simulink model "walec_ostroslup_simulink"  (R2025b)
settings: Solver=FixedStepAuto  StartTime=0.0  StopTime=100  FixedStep=0.0001  RelTol=1e-3
values from neighbouring files (symbols this model uses):
  A2 = 1.47044    [PA_Lab4_walec_ostroslup.m]
  B2 = 4.08042    [PA_Lab4_walec_ostroslup.m]
  C1 = 1.8257    [PA_Lab4_walec_ostroslup.m]
  C2 = 0.745356    [PA_Lab4_walec_ostroslup.m]
  dw = 0.1    [PA_Lab4_walec_ostroslup.m]
  h10 = (qwe0/C1)^2    [PA_Lab4_walec_ostroslup.m]
  H2 = 10    [PA_Lab4_walec_ostroslup.m]
  h20 = 0.5*H2    (= 5)    [PA_Lab4_walec_ostroslup.m]
  kr = 1.2*T_nl/(k_nl*To_nl)    [PA_Lab4_walec_ostroslup.m]
  qwe0 = C2*sqrt(h20)    [PA_Lab4_walec_ostroslup.m]
  R1 = 1.9544    [PA_Lab4_walec_ostroslup.m]
settings Model: Creator=Matadoo  LastModifiedBy=wystr

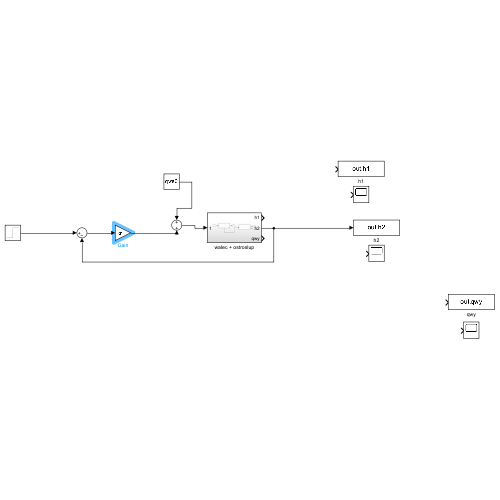
[thumbnail: Simulink's stored preview of the top-level diagram]
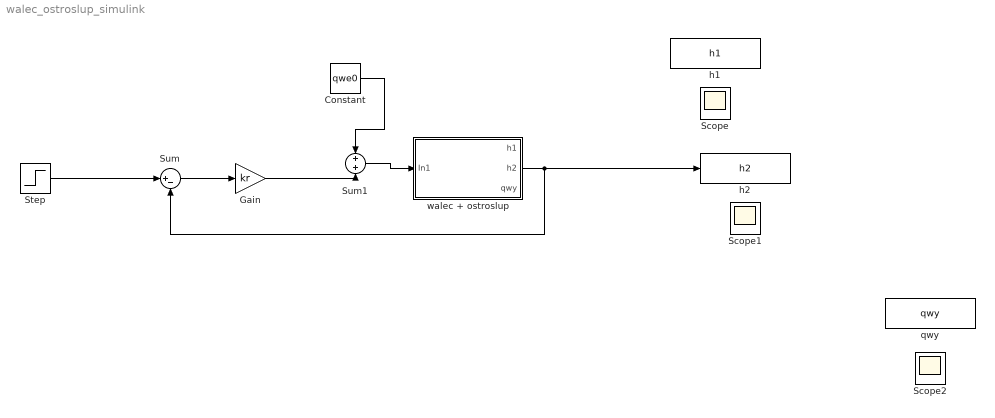
== system walec_ostroslup_simulink ==
  Constant : Constant  Value=qwe0
  Gain : Gain  Gain=kr
  Scope : Scope
      settings: ActiveDisplayYMinimum=-1  ActiveDisplayYMaximum=1
  Scope1 : Scope
      settings: ActiveDisplayYMinimum=0.54521  ActiveDisplayYMaximum=9.07763
  Scope2 : Scope
      settings: ActiveDisplayYMinimum=-1  ActiveDisplayYMaximum=1  DataLoggingVariableName=ScopeData2
  Step : Step  Time=0  Before=h20  After=h20 + dw  SampleTime=0
  Sum : Sum  Inputs=|+-
  Sum1 : Sum  Inputs=+|+
  h1 : ToWorkspace  VariableName=h1  SaveFormat=Timeseries  SampleTime=-1
      settings: Save2DSignal=2-D array (concatenate along first dimension)
  h2 : ToWorkspace  VariableName=h2  SaveFormat=Timeseries  SampleTime=-1
      settings: Save2DSignal=2-D array (concatenate along first dimension)
  qwy : ToWorkspace  VariableName=qwy  SaveFormat=Timeseries  SampleTime=-1
      settings: Save2DSignal=2-D array (concatenate along first dimension)
  walec + ostroslup : Subsystem
  wires:
  walec + ostroslup/2(h2) -> h2/1, Sum/2
  Step/1 -> Sum/1
  Sum/1 -> Gain/1
  Constant/1 -> Sum1/1
  Gain/1 -> Sum1/2
  Sum1/1 -> walec + ostroslup/1(In1)

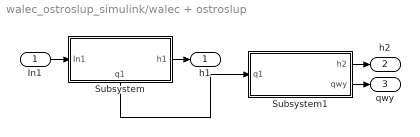
== system walec_ostroslup_simulink/walec + ostroslup ==
  In1 : Inport
  Subsystem : Subsystem
      settings: PortSchema="{\"entries\":[{\"content\":{\"sides\":[{\"content\":{\"connectorIds\":[\"In1\"]},\"type\":\"ConnectorPlacement.EquallySpacedRectSide\",\"uuid\":\"ef9d34a5-cff8-451d-8a8e-ad43d62a4229\"},{\"content\":{\"connectorIds\":[\"Out1\"],\"side\":\"RIGHT\"},\"type\":\"ConnectorPlacement.EquallySpacedRectSide\",\"uuid\":\"a0647498-08a7-49d7-b729-cb433a3947bd\"},{\"content\":{\"side\":\"TOP\"},\"type\":\"ConnectorPlacement.EquallySpacedRectSide\",\"uuid\":\"e54223c9-a9e4-45b8-9f51-507c5557501a\"},{\"content\":{\"connectorIds\":[\"Out2\"],\"side\":\"BOTTOM\"},\"type\":\"ConnectorPlacement.EquallySpacedRectSide\",\"uuid\":\"7d5bf5b3-bf67-4990-a720-c5a5b654a001\"}]},\"type\":\"ConnectorPlacement.EquallySpacedConnector\",\"uuid\":\"879e1674-e5d1-4532-ab14-c8e474c4df17\"}],\"packageUris\":[\"http://schema.mathworks.com/mf0/Connector/R2020b\"],\"version\":\"1.0\"}"
  Subsystem1 : Subsystem
  h1 : Outport
  h2 : Outport  Port=2
  qwy : Outport  Port=3
  wires:
  Subsystem1/1(h2) -> h2/1
  Subsystem1/2(qwy) -> qwy/1
  Subsystem/2(q1) -> Subsystem1/1(q1)
  In1/1 -> Subsystem/1(In1)
  Subsystem/1(h1) -> h1/1

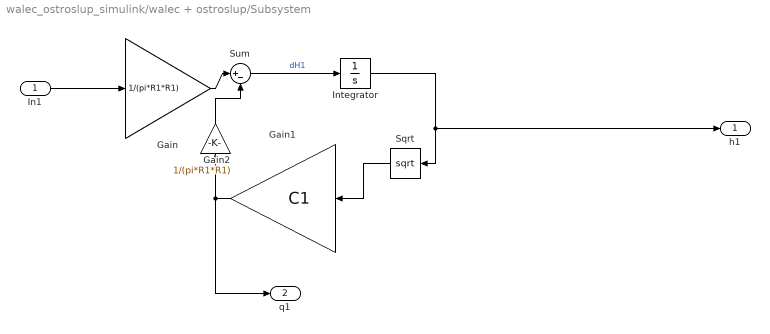
== system walec_ostroslup_simulink/walec + ostroslup/Subsystem ==
  In1 : Inport
  Gain : Gain  Gain=1/(pi*R1*R1)
  Gain1 : Gain  Gain=C1
  Gain2 : Gain  Gain=1/(pi*R1*R1)
  Integrator : Integrator  InitialCondition=h10
  Sqrt : Sqrt
  Sum : Sum  Inputs=|+-
  h1 : Outport
  q1 : Outport  Port=2
  wires:
  Gain/1 -> Sum/1
  Integrator/1 -> h1/1, Sqrt/1
  Sqrt/1 -> Gain1/1
  Gain1/1 -> Gain2/1, q1/1
  Sum/1 -> Integrator/1  "dH1"
  In1/1 -> Gain/1
  Gain2/1 -> Sum/2

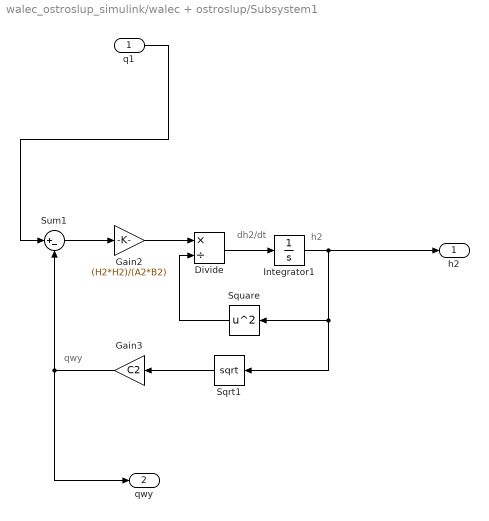
== system walec_ostroslup_simulink/walec + ostroslup/Subsystem1 ==
  note: qwy
  note: dh2/dt
  note: h2
  q1 : Inport
  Divide : Product  Inputs=*/
  Gain2 : Gain  Gain=(H2*H2)/(A2*B2)
  Gain3 : Gain  Gain=C2
  Integrator1 : Integrator  InitialCondition=h20
  Sqrt1 : Sqrt
  Square : Math  Operator=square
  Sum1 : Sum  Inputs=|+-
  h2 : Outport
  qwy : Outport  Port=2
  wires:
  Sum1/1 -> Gain2/1
  Gain3/1 -> qwy/1, Sum1/2
  Square/1 -> Divide/2
  Divide/1 -> Integrator1/1
  Gain2/1 -> Divide/1
  Integrator1/1 -> h2/1, Sqrt1/1, Square/1
  q1/1 -> Sum1/1
  Sqrt1/1 -> Gain3/1
